simulink model "ModeloLab4"  (R2026a)
settings: Solver=VariableStepAuto  StopTime=tsim
values from neighbouring files (symbols this model uses):
  A = 0.5    [Aula08_lab.m]    (also in Lab10.m; Lab5_6.m; lab3.m; lab4.m)
  ae0 = 0.6    [Aula08_lab.m]    (also in Lab10.m; Lab5_6.m; lab3.m; lab4.m = 0:0.01:1)
  as0 = 0.5    [Aula08_lab.m]    (also in Lab10.m; Lab5_6.m; lab3.m; lab4.m = 0:0.01:1)
  delta_Ae = 0.1    [lab4_bonitinho.m]
  delta_As = 0.1    [lab4_bonitinho.m]
  g = 9.8    [Aula08_lab.m]    (also in Lab10.m; Lab5_6.m; lab3.m; lab4.m)
  H0 = ((ke*ae0)/(ks*as0*sqrt(2*g)))^2    [Aula08_lab.m]    (also in Lab10.m; Lab5_6.m; lab3.m = H_eq; lab4.m = ((Ke .* ae0) ./ (Ks .* as0 .* sqrt(2*g))).^2)
  Ke = 0.05    [lab3.m]    (also in lab4.m; lab4_bonitinho.m)
  Ks = 0.015    [lab3.m]    (also in lab4.m; lab4_bonitinho.m)
  tsim = 500    [Aula08_lab.m]    (also in Lab10.m = 1000; Lab5_6.m = 2400; lab4_bonitinho.m = 2400; lab5.m = 200)
libraries: cstblocks_lti x2

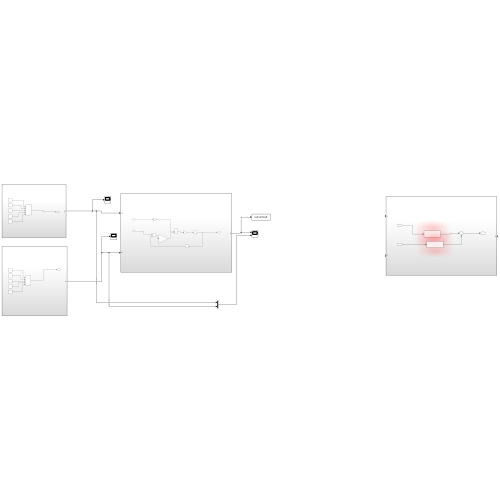
[thumbnail: Simulink's stored preview of the top-level diagram]
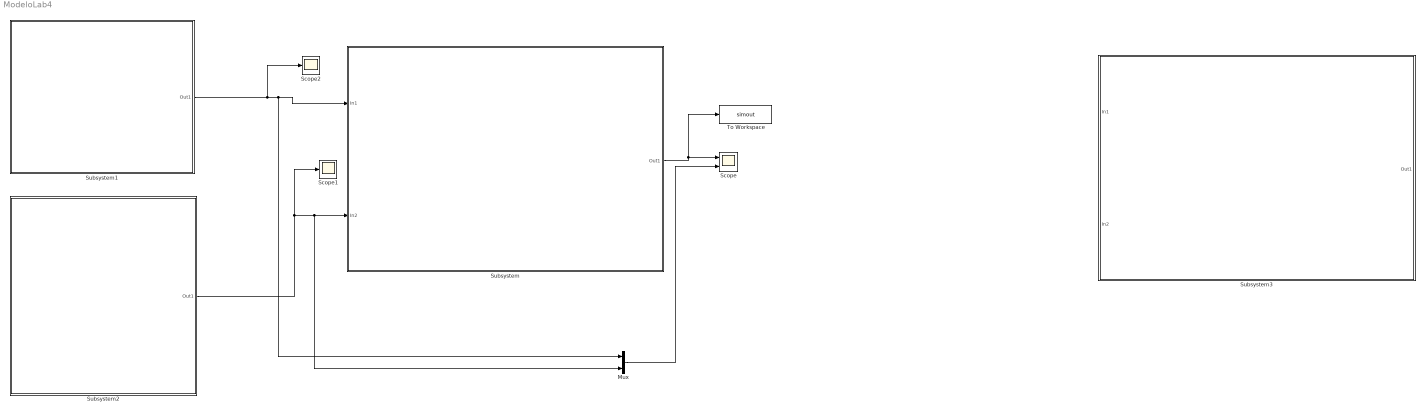
== system ModeloLab4 ==
  Mux : Mux  Inputs=2
  Scope : Scope  NumInputPorts=2
      settings: ActiveDisplayYMinimum=-0.54604239344003869  ActiveDisplayYMaximum=2.108947341956585
  Scope1 : Scope
      settings: ActiveDisplayYMinimum=-0.09127440058818892  ActiveDisplayYMaximum=2.0929922252696578
  Scope2 : Scope
      settings: ActiveDisplayYMinimum=-0.09127440058818892  ActiveDisplayYMaximum=2.0929922252696578  DataLoggingVariableName=ScopeData2
  Subsystem : Subsystem
  Subsystem1 : Subsystem
  Subsystem2 : Subsystem
  Subsystem3 : Subsystem
  To Workspace : ToWorkspace  VariableName=simout  SaveFormat=Timeseries  SampleTime=-1
  wires:
  Subsystem/1(Out1) -> To Workspace/1, Scope/1
  Subsystem2/1(Out1) -> Scope1/1, Mux/2, Subsystem/2(In2)
  Subsystem1/1(Out1) -> Scope2/1, Mux/1, Subsystem/1(In1)
  Mux/1 -> Scope/2

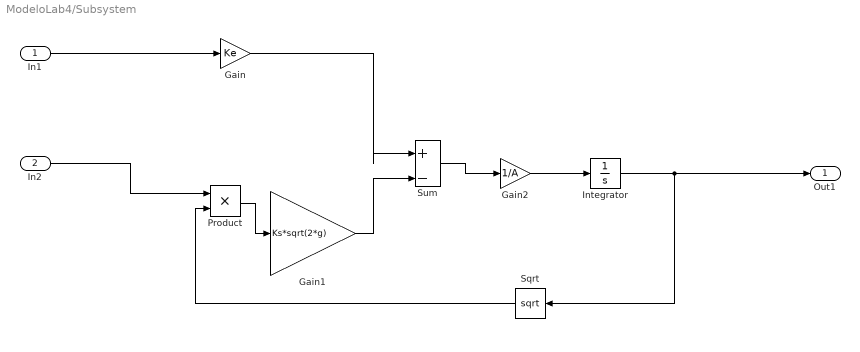
== system ModeloLab4/Subsystem ==
  In1 : Inport
  In2 : Inport  Port=2
  Gain : Gain  Gain=Ke
  Gain1 : Gain  Gain=Ks*sqrt(2*g)
  Gain2 : Gain  Gain=1/A
  Integrator : Integrator  InitialCondition=H0
  Product : Product
  Sqrt : Sqrt
  Sum : Sum  Inputs=|+-
  Out1 : Outport
  wires:
  Gain/1 -> Sum/1
  Product/1 -> Gain1/1
  Gain2/1 -> Integrator/1
  Sum/1 -> Gain2/1
  Sqrt/1 -> Product/2
  In2/1 -> Product/1
  Gain1/1 -> Sum/2
  Integrator/1 -> Out1/1, Sqrt/1
  In1/1 -> Gain/1

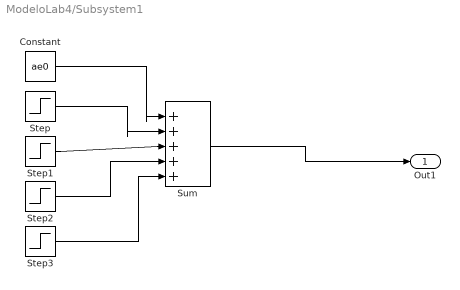
== system ModeloLab4/Subsystem1 ==
  Constant : Constant  Value=ae0
  Step : Step  Time=0  FinalValue=delta_Ae  SampleTime=0
  Step1 : Step  Time=(1/8)*tsim  FinalValue=-delta_Ae  SampleTime=0
  Step2 : Step  Time=(2/8)*tsim  FinalValue=-delta_Ae  SampleTime=0
  Step3 : Step  Time=(3/8)*tsim  FinalValue=delta_Ae  SampleTime=0
  Sum : Sum  Inputs=|+++++
  Out1 : Outport
  wires:
  Sum/1 -> Out1/1
  Step1/1 -> Sum/3
  Step3/1 -> Sum/5
  Step/1 -> Sum/2
  Step2/1 -> Sum/4
  Constant/1 -> Sum/1

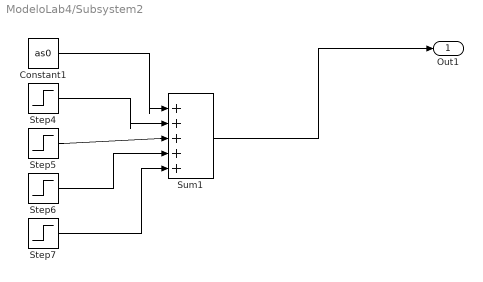
== system ModeloLab4/Subsystem2 ==
  Constant1 : Constant  Value=as0
  Step4 : Step  Time=( 4/8)*tsim  FinalValue=delta_As  SampleTime=0
  Step5 : Step  Time=(5/8)*tsim  FinalValue=-delta_As  SampleTime=0
  Step6 : Step  Time=(6/8)*tsim  FinalValue=-delta_As  SampleTime=0
  Step7 : Step  Time=(7/8)*tsim  FinalValue=delta_As  SampleTime=0
  Sum1 : Sum  Inputs=|+++++
  Out1 : Outport
  wires:
  Constant1/1 -> Sum1/1
  Step5/1 -> Sum1/3
  Step4/1 -> Sum1/2
  Step6/1 -> Sum1/4
  Step7/1 -> Sum1/5
  Sum1/1 -> Out1/1

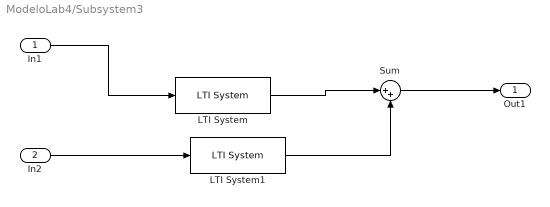
== system ModeloLab4/Subsystem3 ==
  In1 : Inport
  In2 : Inport  Port=2
  LTI System : cstblocks_lti/LTI System  sys=G  IC=[]  PadeOrder=0
      settings: LibrarySourceBlock=cstblocks/LTI System
  LTI System1 : cstblocks_lti/LTI System  sys=Gas  IC=[]  PadeOrder=0
      settings: LibrarySourceBlock=cstblocks/LTI System
  Sum : Sum  Inputs=|++
  Out1 : Outport
  wires:
  In1/1 -> LTI System/1
  In2/1 -> LTI System1/1
  LTI System1/1 -> Sum/2
  LTI System/1 -> Sum/1
  Sum/1 -> Out1/1
